simulink library "SCF_Custom_Forces_lib"  (R2025a)
settings: Solver=VariableStepAuto  StartTime=0.0  StopTime=10.0  RelTol=1e-3
libraries: nesl_utility x6, simulink x1, sm_lib x1
Description:
  | Copyright 2026 The MathWorks, Inc.
settings Model: Creator=smiller  LastModifiedBy=smiller

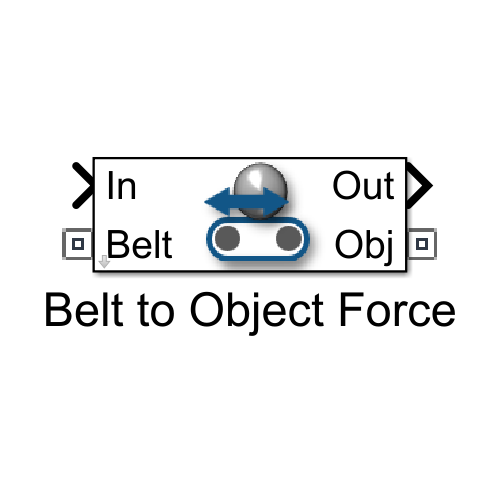
[thumbnail: Simulink's stored preview of the top-level diagram]
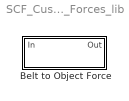
== system SCF_Custom_Forces_lib ==
  Belt to Object Force : Subsystem  mask(Moving Belt to Object Force){k_collision=1e6, d_collision=1e3*10, d_width=1e-3, muk=0.3, mus=0.5, vth=1e-2}
      mask prompts: k_collision "Stiffness Coefficient (N/m)"; d_collision "Damping Coefficient (N/(m/s))"; d_width "Transition Region Width (m)"; muk "Coefficient of Kinetic Friction"; mus "Coefficient of Static Friction"; vth "Velocity Threshold"
      mask help:
      | This subsystem models contact forces between an object and a conveyor belt.  The conveyor belt moves at the speed specified by the input signal in m/s.  The speed and affects upper and lower surfaces of the belt as well as the ends.
      |
      | Geometry connected to Belt port is the for the belt which moves.  The x-axis of the reference frame for the geometry will be the direction of travel for the belt.
      |
      | Geometry connected to the Obj port is the geometry for the object on the belt.  This can be 3D solid geometry (sphere, etc.) or a point cloud.
      |
      | Output signal is a bus with intermediate calculations and total force.
      mask TypeOptions k_collision:
      | Custom
      | Force
      | Law/k_collision
      mask TypeOptions d_collision:
      | Custom
      | Force
      | Law/d_collision
      mask TypeOptions d_width:
      | Custom
      | Force
      | Law/d_width
      mask TypeOptions muk:
      | Custom
      | Force
      | Law/muk
      mask TypeOptions mus:
      | Custom
      | Force
      | Law/mus
      mask TypeOptions vth:
      | Custom
      | Force
      | Law/vth
      mask DialogControl cont_contact Prompt: Contact
      mask DialogControl cont_normalForce Prompt: Normal Force
      mask DialogControl cont_frictionForce Prompt: Friction Force
      mask Display: image('SFC_Belt_to_Object_IMAGE.png');

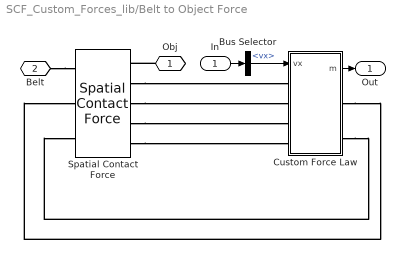
== system SCF_Custom_Forces_lib/Belt to Object Force ==
  In : Inport
  Bus Selector : BusSelector  OutputSignals=vx
  Custom Force Law : Subsystem  mask(Moving Belt to Object Force Law){k_collision=k_collision, d_collision=d_collision, d_width=d_width, mus=mus, muk=muk, vth=vth}
      mask prompts: k_collision "Stiffness Coefficient (N/m)"; d_collision "Damping Coefficient (N/(m/s))"; d_width "Transition Region Width (m)"; mus "Coefficient of Static Friction"; muk "Coefficient of Kinetic Friction"; vth "Velocity Threshold"
      mask help:
      | This subsystem calculates the contact forces between an object and a conveyor belt.  The conveyor belt moves at the speed specified by the input signal in m/s.
      |
      | Quantities for this force law (separation, separation velocity, tangential velocity, and contact frame rotation matrix) must be obtained from the Spatial Contact Force block so that the resulting forces can be calculated in the correct frame.
      |
      | The vx input is the speed of the belt surface along the positive x-axis of the reference frame for the belt contact geometry.
      |
      | Output signal is a bus with intermediate calculations and total force.
      mask TypeOptions k_collision: Normal Force/k_collision
      mask TypeOptions d_collision: Normal Force/d_collision
      mask TypeOptions d_width: Normal Force/d_width
      mask TypeOptions mus:
      | Friction Law
      | /mus
      mask TypeOptions muk:
      | Friction Law
      | /muk
      mask TypeOptions vth:
      | Friction Law
      | /vth
      mask DialogControl cont_contact Prompt: Contact
      mask DialogControl cont_normalForce Prompt: Normal Force
      mask DialogControl cont_frictionForce Prompt: Friction Force
  Spatial Contact Force : sm_lib/Forces and Torques/Spatial Contact Force  SenseSeparationDistance=off  NormalForceType=ProvidedByInput  NormalStiffness=1e6  NormalStiffnessUnits=N/m  NormalDamping=1e3  NormalDampingUnits=N/(m/s)  NormalTransitionRegionWidth=1e-4  NormalTransitionRegionWidthUnits=m  FrictionType=ProvidedByInput  CoefficientOfStaticFriction=0.5  CoefficientOfDynamicFriction=0.3  FrictionalCriticalVelocity=1e-3  FrictionalCriticalVelocityUnits=m/s  SenseContactSignal=off  SensePenetrationDepth=on  SenseNormalVelocity=on  SenseTangentialVelocity=on  SensingForceTorqueDirection=BaseOnFollower  SensingForceTorqueResolutionFrame=ContactFrame  SenseNormalForce=off  SenseNormalForceMagnitude=off  SenseNormalTorque=off  SenseFrictionalForce=off  SenseFrictionalForceMagnitude=off  SenseFrictionalTorque=off  SenseTotalForce=off  SenseTotalTorque=off  SenseContactBaseRotation=on  SenseContactBaseTranslation=off  SenseContactFollowerRotation=off  SenseContactFollowerTranslation=off  ZeroCrossDetectContactStartAndEnd=off
  Obj : PMIOPort  Side=Right
  Belt : PMIOPort  Port=2  Side=Left
  Out : Outport
  wires:
  Bus Selector/1 -> Custom Force Law/1(vx)  "<vx>"
  In/1 -> Bus Selector/1
  Custom Force Law/1(m) -> Out/1
  connections:
  Spatial Contact Force/RConn2 -- Custom Force Law/LConn1
  Custom Force Law/RConn2 -- Spatial Contact Force/LConn3
  Custom Force Law/RConn1 -- Spatial Contact Force/LConn2
  Obj/RConn1 -- Spatial Contact Force/RConn1
  Belt/RConn1 -- Spatial Contact Force/LConn1
  Spatial Contact Force/RConn3 -- Custom Force Law/LConn2
  Spatial Contact Force/RConn4 -- Custom Force Law/LConn3
  Spatial Contact Force/RConn5 -- Custom Force Law/LConn4

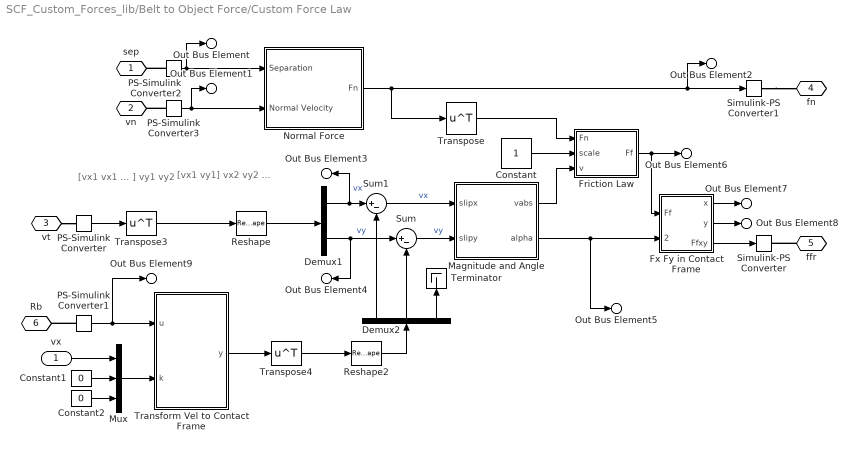
== system SCF_Custom_Forces_lib/Belt to Object Force/Custom Force Law ==
  note: [vx1 vx1 ... ]
      |  vy1 vy2
  note: [vx1 vy1]
      |  vx2 vy2
      |  ...
  vx : Inport
  Constant : Constant
  Constant1 : Constant  Value=0
  Constant2 : Constant  Value=0
  Demux1 : Demux  Outputs=2
  Demux2 : Demux  Outputs=3
  "Friction Law " : Subsystem  VariantControl=Stick_Slip_C  mask(Stick-Slip Friction, Continuous){muk=muk, mus=mus, vth=vth}
      mask prompts: muk "Coefficient of Kinetic Friction"; mus "Coefficient of Static Friction"; vth "Velocity Threshold"
      mask help: Implements a continuous stick-slip friction model. Smaller velocity threshold is closer to reality but results in a numerically stiffer system.
  Fx Fy in Contact Frame : Subsystem
  Magnitude and Angle : Subsystem
  Mux : Mux  Inputs=3
  Normal Force : Subsystem  mask{k_collision=k_collision, d_collision=d_collision, d_width=d_width}
      mask prompts: k_collision "Stiffness Coefficient (N/m)"; d_collision "Damping Coefficient (N/(m/s))"; d_width "Transition Region Width (m)"
  PS-Simulink Converter{,1..3} (4 alike) : nesl_utility/PS-Simulink Converter  PhysicalDomain=network_engine_domain  SubClassName=ps_output  LeftPortType=input  RightPortType=output  PseudoPeriodic=off  Frequencies=[]  VectorFormat=inherit  Unit=inherit  AffineConversion=off
  Reshape : Reshape
  Reshape2 : Reshape
  Simulink-PS Converter : nesl_utility/Simulink-PS Converter  PhysicalDomain=network_engine_domain  SubClassName=ps_input  LeftPortType=input  RightPortType=output  PseudoPeriodic=off  Frequencies=[]  NoiseDistribution=none  NoiseParameters=[]  Unit=1  AffineConversion=off  FilteringAndDerivatives=provide  SimscapeFilterOrder=1  InputFilterTimeConstant=0.001  UdotUserProvided=0
  Simulink-PS Converter1 : nesl_utility/Simulink-PS Converter  PhysicalDomain=network_engine_domain  SubClassName=ps_input  LeftPortType=input  RightPortType=output  PseudoPeriodic=off  Frequencies=[]  NoiseDistribution=none  NoiseParameters=[]  Unit=1  AffineConversion=off  FilteringAndDerivatives=provide  SimscapeFilterOrder=1  InputFilterTimeConstant=0.001  UdotUserProvided=0
  Sum : Sum  Inputs=|+-
  Sum1 : Sum  Inputs=|+-
  Terminator : Terminator
  Transform Vel to Contact Frame : MATLAB Function  TreatAsAtomicUnit=on
  Transpose : Math  Operator=transpose
  Transpose3 : Math  Operator=transpose
  Transpose4 : Math  Operator=transpose
  sep : PMIOPort  Side=Left
  vn : PMIOPort  Port=2  Side=Left
  vt : PMIOPort  Port=3  Side=Left
  fn : PMIOPort  Port=4  Side=Right
  ffr : PMIOPort  Port=5  Side=Right
  Rb : PMIOPort  Port=6  Side=Left
  Out Bus Element : Outport  PortName=m  Element=sep
  Out Bus Element1 : Outport  PortName=m  Element=vn
  Out Bus Element2 : Outport  PortName=m  Element=fn
  Out Bus Element3 : Outport  PortName=m  Element=vt.x
  Out Bus Element4 : Outport  PortName=m  Element=vt.y
  Out Bus Element5 : Outport  PortName=m  Element=alpha
  Out Bus Element6 : Outport  PortName=m  Element=Ff.mag
  Out Bus Element7 : Outport  PortName=m  Element=Ff.x
  Out Bus Element8 : Outport  PortName=m  Element=Ff.y
  Out Bus Element9 : Outport  PortName=m  Element=Rb
  wires:
  "Friction Law "/1(Ff) -> Out Bus Element6/1, Fx Fy in Contact Frame/1(Ff)
  Magnitude and Angle/1(vabs) -> "Friction Law "/3(v)
  Normal Force/1(Fn) -> Transpose/1, Out Bus Element2/1, Simulink-PS Converter1/1
  PS-Simulink Converter2/1 -> Normal Force/1(Separation), Out Bus Element/1
  Fx Fy in Contact Frame/3(Ffxy) -> Simulink-PS Converter/1
  Constant/1 -> "Friction Law "/2(scale)
  Reshape/1 -> Demux1/1
  Transpose/1 -> "Friction Law "/1(Fn)
  Sum1/1 -> Magnitude and Angle/1(slipx)  "vx"
  vx/1 -> Mux/1
  Sum/1 -> Magnitude and Angle/2(slipy)  "vy"
  PS-Simulink Converter/1 -> Transpose3/1
  Transform Vel to Contact Frame/1(y) -> Transpose4/1
  Reshape2/1 -> Demux2/1
  Transpose4/1 -> Reshape2/1
  Constant1/1 -> Mux/2
  Mux/1 -> Transform Vel to Contact Frame/2(k)
  Transpose3/1 -> Reshape/1
  Magnitude and Angle/2(alpha) -> Out Bus Element5/1, Fx Fy in Contact Frame/2(alpha)
  Demux1/1 -> Out Bus Element3/1, Sum1/1  "vx"
  Demux1/2 -> Out Bus Element4/1, Sum/1  "vy"
  Demux2/1 -> Sum1/2
  Demux2/2 -> Sum/2
  Constant2/1 -> Mux/3
  Demux2/3 -> Terminator/1
  PS-Simulink Converter1/1 -> Out Bus Element9/1, Transform Vel to Contact Frame/1(u)
  PS-Simulink Converter3/1 -> Out Bus Element1/1, Normal Force/2(Normal Velocity)
  Fx Fy in Contact Frame/1(x) -> Out Bus Element7/1
  Fx Fy in Contact Frame/2(y) -> Out Bus Element8/1
  connections:
  vt/RConn1 -- PS-Simulink Converter/LConn1
  PS-Simulink Converter2/LConn1 -- sep/RConn1
  PS-Simulink Converter3/LConn1 -- vn/RConn1
  Simulink-PS Converter1/RConn1 -- fn/RConn1
  ffr/RConn1 -- Simulink-PS Converter/RConn1
  PS-Simulink Converter1/LConn1 -- Rb/RConn1

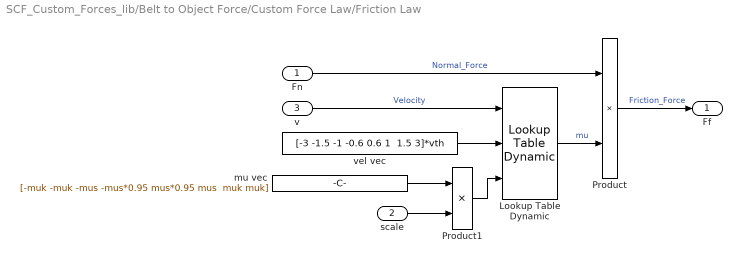
== system SCF_Custom_Forces_lib/Belt to Object Force/Custom Force Law/Friction Law  ==
  Fn : Inport
  scale : Inport  Port=2
  v : Inport  Port=3
  Lookup Table Dynamic : simulink/Lookup Tables/Lookup Table Dynamic  LookUpMeth=Interpolation-Use End Values  OutDataType=fixdt('double')  OutScaling=[]  OutputDataTypeScalingMode=Specify via dialog  OutDataTypeStr=double  DoSatur=off
  Product : Product  RndMeth=Zero
  Product1 : Product
  mu vec : Constant  Value="[-muk -muk -mus -mus*0.95 mus*0.95 mus  muk muk]"
  vel vec : Constant  Value="[-3 -1.5 -1 -0.6 0.6 1  1.5 3]*vth"
  Ff : Outport  VectorParamsAs1DForOutWhenUnconnected=off
  wires:
  Product/1 -> Ff/1  "Friction_Force"
  v/1 -> Lookup Table Dynamic/1  "Velocity"
  Fn/1 -> Product/1  "Normal_Force"
  vel vec/1 -> Lookup Table Dynamic/2
  mu vec/1 -> Product1/1
  Product1/1 -> Lookup Table Dynamic/3
  Lookup Table Dynamic/1 -> Product/2  "mu"
  scale/1 -> Product1/2

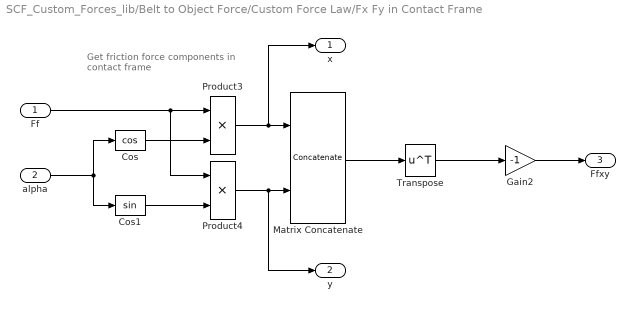
== system SCF_Custom_Forces_lib/Belt to Object Force/Custom Force Law/Fx Fy in Contact Frame ==
  note: Get friction force components
      | in contact frame
  Ff : Inport
  alpha : Inport  Port=2
  Cos : Trigonometry  Operator=cos
  Cos1 : Trigonometry
  Gain2 : Gain  Gain=-1
  Matrix Concatenate : Concatenate  Mode=Multidimensional array  ConcatenateDimension=2
  Product3 : Product
  Product4 : Product
  Transpose : Math  Operator=transpose
  x : Outport
  y : Outport  Port=2
  Ffxy : Outport  Port=3
  wires:
  Ff/1 -> Product3/1, Product4/1
  Matrix Concatenate/1 -> Transpose/1
  Product3/1 -> x/1, Matrix Concatenate/1
  Product4/1 -> y/1, Matrix Concatenate/2
  alpha/1 -> Cos1/1, Cos/1
  Cos/1 -> Product3/2
  Cos1/1 -> Product4/2
  Transpose/1 -> Gain2/1
  Gain2/1 -> Ffxy/1

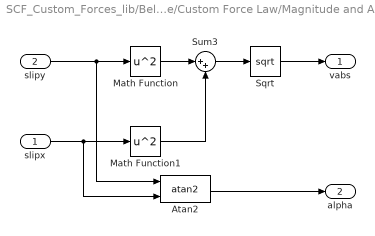
== system SCF_Custom_Forces_lib/Belt to Object Force/Custom Force Law/Magnitude and Angle ==
  slipx : Inport
  slipy : Inport  Port=2
  Atan2 : Trigonometry  Operator=atan2
  Math Function : Math  Operator=square  SignedPower=on
  Math Function1 : Math  Operator=square  SignedPower=on
  Sqrt : Sqrt
  Sum3 : Sum  Inputs=|++
  vabs : Outport  VectorParamsAs1DForOutWhenUnconnected=off
  alpha : Outport  Port=2  VectorParamsAs1DForOutWhenUnconnected=off
  wires:
  Math Function/1 -> Sum3/1
  slipx/1 -> Atan2/2, Math Function1/1
  slipy/1 -> Atan2/1, Math Function/1
  Math Function1/1 -> Sum3/2
  Sqrt/1 -> vabs/1
  Sum3/1 -> Sqrt/1
  Atan2/1 -> alpha/1

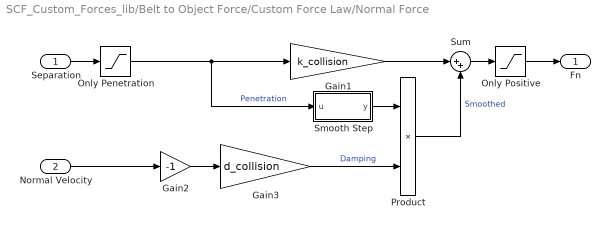
== system SCF_Custom_Forces_lib/Belt to Object Force/Custom Force Law/Normal Force ==
  Separation : Inport
  Normal Velocity : Inport  Port=2
  Gain1 : Gain  Gain=k_collision
  Gain2 : Gain  Gain=-1
  Gain3 : Gain  Gain=d_collision  SaturateOnIntegerOverflow=on  OutDataTypeStr=Inherit: Same as input  ParamDataTypeStr=Inherit: Same as input
  Only Penetration : Saturate  UpperLimit=inf  LowerLimit=0
  Only Positive : Saturate  UpperLimit=inf  LowerLimit=0  ZeroCross=off
  Product : Product  RndMeth=Zero
  Smooth Step : Subsystem  mask(Smooth step function){step_start=0, step_finish=d_width, min_out=0, max_out=1}
      mask prompts: step_start "Start Step (u)"; step_finish "Finish Step (u)"; min_out "Minimum output (y)"; max_out "Maximum output (y)"
      mask help:
      | Smooth step function
      | y=3u^2-2u^3
      | Input and output ranges scaled by parameters.
      settings: AttributesFormatString=%<step_start> to %<step_finish>
  Sum : Sum  Inputs=|++
  Fn : Outport
  wires:
  Separation/1 -> Only Penetration/1
  Only Positive/1 -> Fn/1
  Sum/1 -> Only Positive/1
  Gain1/1 -> Sum/1
  Smooth Step/1(y) -> Product/1
  Only Penetration/1 -> Smooth Step/1(u), Gain1/1  "Penetration"
  Gain3/1 -> Product/2  "Damping"
  Normal Velocity/1 -> Gain2/1
  Product/1 -> Sum/2  "Smoothed"
  Gain2/1 -> Gain3/1

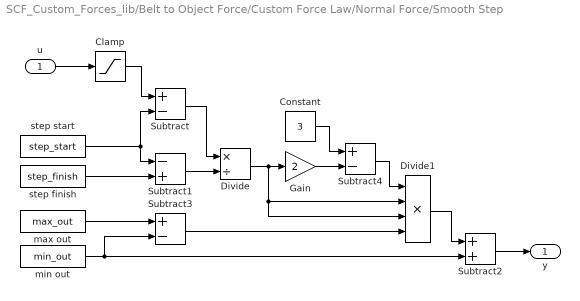
== system SCF_Custom_Forces_lib/Belt to Object Force/Custom Force Law/Normal Force/Smooth Step ==
  u : Inport
  Clamp : Saturate  UpperLimit=step_finish  LowerLimit=step_start
  Constant : Constant  Value=3
  Divide : Product  Inputs=*/
  Divide1 : Product  Inputs=****
  Gain : Gain  Gain=2
  Subtract : Sum  Inputs=+-
  Subtract1 : Sum  Inputs=-+
  Subtract2 : Sum
  Subtract3 : Sum  Inputs=+-
  Subtract4 : Sum  Inputs=+-
  max out : Constant  Value=max_out
  min out : Constant  Value=min_out
  step finish : Constant  Value=step_finish
  step start : Constant  Value=step_start
  y : Outport  VectorParamsAs1DForOutWhenUnconnected=off
  wires:
  step start/1 -> Subtract1/1, Subtract/2
  u/1 -> Clamp/1
  Subtract1/1 -> Divide/2
  Divide/1 -> Gain/1, Divide1/2, Divide1/3
  Subtract/1 -> Divide/1
  Subtract2/1 -> y/1
  Constant/1 -> Subtract4/1
  min out/1 -> Subtract2/2, Subtract3/2
  max out/1 -> Subtract3/1
  Clamp/1 -> Subtract/1
  step finish/1 -> Subtract1/2
  Divide1/1 -> Subtract2/1
  Gain/1 -> Subtract4/2
  Subtract4/1 -> Divide1/1
  Subtract3/1 -> Divide1/4

== matlab function SCF_Custom_Forces_lib/Belt to Object Force/Custom Force Law/Transform Vel to Contact Frame ==
  data: u input; y output; k input
function y = fcn(u, k)

[~,~,p] = size(u);

y =zeros(3,p);

for i = 1:p
    % Extract the rotation matrix
    mtx = u(:,:,i);
    % Premultiply the vector by the transpose
    % of the rotation matrix to express k in 
    % the desired coordinate system.
    y(:,i) = mtx'*k;
end
